simulink model "os_supervisor_chart"  (R2026b)
settings: Solver=FixedStepDiscrete  StopTime=2  FixedStep=0.001
model workspace (MAT data in the model file):
  limits = [100; 200; 500; 1000; 5; 20]
  stimulus = timeseries
  stimulus.Name = 'unnamed'
  stimulus.DataInfo = tsdata.datametadata
  stimulus.DataInfo.Interpolation = tsdata.interpolation
  stimulus.DataInfo.Interpolation.Fhandle : function handle (value not decoded)
  stimulus.DataInfo.Interpolation.Name = 'linear'
  stimulus.TimeInfo = tsdata.timemetadata
  stimulus.TimeInfo.Length = 2101
  stimulus.TimeInfo.DuplicateTimes = 0
  stimulus.TimeInfo.Time_ = [0 0.001 0.002 0.003 0.004 0.005 0.006 0.007 0.008 0.009 0.01 0.011 ... (2101 elements, 2101x1)]
  stimulus.TimeInfo.Initialized = 1
  stimulus.QualityInfo = tsdata.qualmetadata
  stimulus.Data_ = [0 1 2 3 4 5 6 7 8 9 10 11 ... (10505 elements, 2101x5)]
settings Model: Creator=Contributor  LastModifiedBy=Contributor
settings DataIOCC: SaveOutput=off

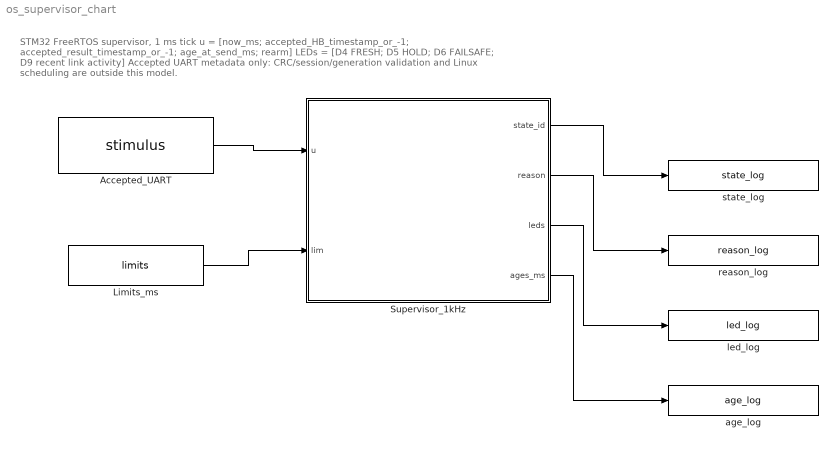
== system os_supervisor_chart ==
  note: STM32 FreeRTOS supervisor, 1 ms tick
      | u = [now_ms; accepted_HB_timestamp_or_-1; accepted_result_timestamp_or_-1; age_at_send_ms; rearm]
      | LEDs = [D4 FRESH; D5 HOLD; D6 FAILSAFE; D9 recent link activity]
      | Accepted UART metadata only: CRC/session/generation validation and Linux scheduling are outside this model.
  Accepted_UART : FromWorkspace  VariableName=stimulus  SampleTime=0.001  Interpolate=off  OutputAfterFinalValue=Holding final value
  Limits_ms : Constant  Value=limits
  Supervisor_1kHz : Stateflow chart  TreatAsAtomicUnit=on
  age_log : ToWorkspace  VariableName=age_log  SaveFormat=Timeseries  SampleTime=-1
  led_log : ToWorkspace  VariableName=led_log  SaveFormat=Timeseries  SampleTime=-1
  reason_log : ToWorkspace  VariableName=reason_log  SaveFormat=Timeseries  SampleTime=-1
  state_log : ToWorkspace  VariableName=state_log  SaveFormat=Timeseries  SampleTime=-1
  wires:
  Accepted_UART/1 -> Supervisor_1kHz/1(u)
  Limits_ms/1 -> Supervisor_1kHz/2(lim)
  Supervisor_1kHz/1(state_id) -> state_log/1
  Supervisor_1kHz/2(reason) -> reason_log/1
  Supervisor_1kHz/3(leds) -> led_log/1
  Supervisor_1kHz/4(ages_ms) -> age_log/1

== stateflow chart os_supervisor_chart/Supervisor_1kHz ==
  settings: updateMethod=DISCRETE  sampleTime=0.001  description=Timing abstraction of OS_PLAN and retained firmware: pre-reception deadline checks; explicit healthy rearm; new receptions after rearm.
  state SUPERVISOR
    entry:
    nowMs=u(1); lastHB=0; lastResult=0; ageAtSend=0; epoch=nowMs;
    hasHB=false; hasResult=false; healthySince=-1; activityUntil=-1;
    hbExpired=true; sourceExpired=false; healthy=false;
    heartbeatAge=0; sourceAge=0; leds=zeros(4,1); ages_ms=zeros(2,1);
    during:
    nowMs=u(1);
    heartbeatAge=nowMs-lastHB; sourceAge=nowMs-lastResult+ageAtSend+lim(5);
    hbExpired=~hasHB || heartbeatAge>=lim(1);
    sourceExpired=hasResult && sourceAge>=lim(3);
    if hbExpired || ~hasResult || sourceAge>=lim(2)
    healthySince=-1;
    end
    if u(2)>epoch && u(2)<=nowMs && (~hasHB || u(2)>lastHB)
    lastHB=u(2); hasHB=true; activityUntil=nowMs+lim(6);
    end
    if u(3)>epoch && u(3)<=nowMs && (~hasResult || u(3)>lastResult)
    lastResult=u(3); ageAtSend=u(4); hasResult=true; activityUntil=nowMs+lim(6);
    end
    heartbeatAge=nowMs-lastHB; sourceAge=nowMs-lastResult+ageAtSend+lim(5);
    hbExpired=hbExpired || ~hasHB || heartbeatAge>=lim(1);
    sourceExpired=sourceExpired || (hasResult && sourceAge>=lim(3));
    healthy=hasHB && hasResult && heartbeatAge<lim(1) && sourceAge<lim(2);
    if healthy
    if healthySince<0
    healthySince=nowMs;
    end
    else
    healthySince=-1;
    end
    leds(4)=double(nowMs<activityUntil);
    ages_ms=[heartbeatAge;sourceAge];
    state INIT
      entry:
      state_id=0; reason=0; epoch=nowMs;
      hasHB=false; hasResult=false; healthy=false; healthySince=-1;
      leds(1)=0; leds(2)=0; leds(3)=0;
    state FRESH
      entry:
      state_id=1; reason=1;
      leds(1)=1; leds(2)=0; leds(3)=0;
    state FAILSAFE
      entry:
      state_id=3;
      leds(1)=0; leds(2)=0; leds(3)=1;
    state HOLD
      entry:
      state_id=2; reason=9;
      leds(1)=0; leds(2)=1; leds(3)=0;
    FAILSAFE -> INIT : [u(5)>0 && healthy && healthySince>=0 && nowMs-healthySince>=lim(4)]
    (default) -> INIT
    INIT -> FRESH [order 2] : [healthy && lastHB>epoch && lastResult>epoch]
    HOLD -> FRESH [order 3] : [healthy]
    FRESH -> HOLD [order 3] : [hasResult && sourceAge>=lim(2)]
    INIT -> FAILSAFE [order 1] : [sourceExpired]{reason=10;}
    FRESH -> FAILSAFE [order 1] : [hbExpired]{reason=3;}
    FRESH -> FAILSAFE [order 2] : [sourceExpired]{reason=10;}
    HOLD -> FAILSAFE [order 1] : [hbExpired]{reason=3;}
    HOLD -> FAILSAFE [order 2] : [sourceExpired]{reason=10;}
  (default) -> SUPERVISOR
  data: u input double size=[5 1]; lim input double size=[6 1]; state_id output double size=1; reason output double size=1; leds output double size=[4 1]; ages_ms output double size=[2 1]; lastHB local double size=1; lastResult local double size=1; ageAtSend local double size=1; epoch local double size=1; healthySince local double size=1; nowMs local double size=1; sourceAge local double size=1; heartbeatAge local double size=1; activityUntil local double size=1; hasHB local boolean size=1; hasResult local boolean size=1; hbExpired local boolean size=1; sourceExpired local boolean size=1; healthy local boolean size=1
